simulink model "Inverter_pq_comp_sim"  (R2023b)
settings: Solver=FixedStepDiscrete  StartTime=0.0  StopTime=2  RelTol=1e-3  EnableMultiTasking=on
InitFcn:
  | %% Definition of the parameters
  | 
  | Parameter_Definition
  | 
  | %% Damping
  | 
  | Rd = 3.9;
  | 
  | %% PRes Gains Calculation
  | 
  | % Definicao das grandezas
  | w_cl = 1j*2*pi*1200;  % Phase Crossing Frequency
  | no   = 1;           % Integral Resonant Constant
  | A    = 1;             % Carrier Amplitude
  | 
  | % Kp calculation
  | a0 = 1;
  | a1 = Rd*Cf;
  | b0 = 0;
  | b1 = Lf+Lg;
  | b2 = Rd*Lf*Cf+Rd*Lg*Cf;
  | b3 = Lf*Lg*Cf;
  | 
  | G_lcl = (a1*w_cl+a0)/(b3*w_cl^3+b2*w_cl^2+b1*w_cl+b0);
  | % G_lcl = 1/((Lf+Lg)*w_cl+Rf);
  | 
  | G_PWM = (1/A)*(1-w_cl*Ts/4)/(1+w_cl*Ts/4);
  | 
  | G_wc  = (Vdc/2)*(1/I_base)*G_lcl*G_PWM;
  | 
  | G_wc_abs = abs(G_wc);
  | 
  | Kp = 0.8/G_wc_abs;
  | 
  | % Discretized Controller Gains
  | ressonance_list = [1,5,7];
  | 
  | n_res = length(ressonance_list);
  | a = zeros(2,n_res);
  | b = zeros(2,n_res);
  | Ki_res = zeros(1,n_res);
  | 
  | % for i = 1:n_res
  | %   k = ressonance_list(i);
  | %   Ki_res(i) = (2.2*Kp)/(no*T_gr);
  | %   a(i) = (2*Ki_res(i)*Ts)/(4+((k*w_gr)^2)*Ts^2);
  | %   b(i) = (-8+2*((k*w_gr)^2)*Ts^2)/(4+((k*w_gr)^2)*Ts^2);
  | % end
  | 
  | % wc is the cutoff frequency/damping factor in rad/s
  | wc = 5;
  | 
  | for i = 1:n_res
  |   k = ressonance_list(i);
  |   wk = k * w_gr; % Resonant frequency for this harmonic
  | 
  |   Ki_res(i) = (2.2*Kp)/(0.8*no*T_gr);
  | 
  |   % 1. Calculate the common denominator
  |   den = 4 + 4*wc*Ts + (wk^2)*(Ts^2);
  | ... (+14 lines)
values from neighbouring files (symbols this model uses):
  a1_sogi = single(2*(w0_sogi^2-c_sogi^2)/den0_sogi)    [Parameter_Definition.m]
  a2_sogi = single((c_sogi^2                 - k_sogi*w0_sogi*c_sogi                 + w0_sogi^2)/den0_sogi)    [Parameter_Definition.m]
  bD_sogi = single(k_sogi*w0_sogi*c_sogi/den0_sogi)    [Parameter_Definition.m]
  bQ_sogi = single(k_sogi*w0_sogi^2/den0_sogi)    [Parameter_Definition.m]
  Cdc = 1.5e-3    (= 0.0015)    [Parameter_Definition.m]
  Cf = 5e-6    (= 5e-06)    [Parameter_Definition.m]
  f_gr = 60    [Parameter_Definition.m]
  I_base = S_base/(sqrt(3)*V_gr)    [Parameter_Definition.m]
  Lf = 1e-3    (= 0.001)    [Parameter_Definition.m]
  Lg = 0.5e-3    (= 0.0005)    [Parameter_Definition.m]
  Rdc = 0.1/(2*pi*60*Cdc)    (= 0.176838825658)    [Parameter_Definition.m]
  Rf = 0.1*Xf    (= 0.0376991118431)    [Parameter_Definition.m]
  Rg = 0.1*Xg    (= 0.0188495559215)    [Parameter_Definition.m]
  S_base = S_rated    (= 1000)    [Parameter_Definition.m]
  Ts = 2*(4167)/100e6    (= 8.334e-05)    [Parameter_Definition.m]
  Tstep = Ts/1000    (= 8.334e-08)    [Parameter_Definition.m]
  V_base = sqrt(3)*V_gr    [Parameter_Definition.m]
  V_gr = 127    [Parameter_Definition.m]
  Vdc = 800    [Parameter_Definition.m]
  Vdc_base = Vdc    (= 800)    [Parameter_Definition.m]
  w_gr = 2*pi*f_gr    (= 376.991118431)    [Parameter_Definition.m]
libraries: spsSeriesRLCBranchLib x14, spsIGBTDiodeLib x12, spsCurrentMeasurementLib x6, spsVoltageMeasurementLib x5, c2837xDlib x4, spsACVoltageSourceLib x3, spsGroundLib x3, spsDCVoltageSourceLib x2, spsTriangleGeneratorLib x1, simulink x1, spsThreePhaseBreakerLib x1, sps_lib x1
(part 2 of 2)

== matlab function Inverter_pq_comp_sim/Current Controller/PRes ==
  data: Kp input; a input; b input; errora input; ma output; errorb input; mb output; enable input
function [ma, mb] = PResCurrent(Kp, a, b, errora, errorb, enable)

%Controller modeled in abc frame, considering p.u. values

%%% Variables Definition
%%%%#########################################################
%%%%######################################################### 

nRes = length(a);

max_pu = single(1.0);

%Proportional part variable
%Phase a
persistent pia
    if isempty(pia)
        pia = single(0.0);
    end
%Phase b    
persistent pib
    if isempty(pib)
        pib = single(0.0);
    end 
    
%Resonant parts variables
%Phase a
persistent presa
    if isempty(presa)
        presa = zeros(1,nRes);
    end
persistent presa_1d %1 sample delay
    if isempty(presa_1d)
        presa_1d = zeros(1,nRes);
    end    
persistent presa_2d %2 samples delay
    if isempty(presa_2d)
        presa_2d = zeros(1,nRes);
    end
persistent presOUT_ia
    if isempty(presOUT_ia)
        presOUT_ia = single(0.0);
    end
    
%Phase b
persistent presb
    if isempty(presb)
        presb = zeros(1,nRes);
    end
persistent presb_1d %1 sample delay
    if isempty(presb_1d)
        presb_1d = zeros(1,nRes);
    end    
persistent presb_2d %2 samples delay
    if isempty(presb_2d)
        presb_2d = zeros(1,nRes);
    end
persistent presOUT_ib
    if isempty(presOUT_ib)
        presOUT_ib = single(0.0);
    end

%Error variables
%Phase a
% persistent errora %Actual error
%     if isempty(errora)
%         errora = 0.0;
%     end
persistent errora_0d %Actual error to delay
    if isempty(errora_0d)
        errora_0d = single(0.0);
    end
persistent errora_1d %1 sample delay
    if isempty(errora_1d)
        errora_1d = single(0.0);
    end    
persistent errora_2d %2 sample delay
    if isempty(errora_2d)
        errora_2d = single(0.0);
    end   
%Phase b
% persistent errorb %Actual error
%     if isempty(errorb)
%         errorb = 0.0;
%     end
persistent errorb_0d %Actual error to delay
    if isempty(errorb_0d)
        errorb_0d = single(0.0);
    end
persistent errorb_1d %1 sample delay
    if isempty(errorb_1d)
        errorb_1d = single(0.0);
    end    
persistent errorb_2d %2 sample delay
    if isempty(errorb_2d)
        errorb_2d = single(0.0);
    end

%%% Enable logic
%%%%#########################################################
%%%%#########################################################

if ~enable 
    % Define safe outputs
    ma = single(0.0);
    mb = single(0.0);
    mc = single(0.0);
    
    % Reset history registers for bumpless transfer
    pia = single(0.0); pib = single(0.0);
    
    presa       = zeros(1,nRes);
    presa_1d    = zeros(1,nRes);
    presa_2d    = zeros(1,nRes);
    presOUT_ia  = single(0.0);
    
    presb       = zeros(1,nRes);
    presb_1d    = zeros(1,nRes);
    presb_2d    = zeros(1,nRes);
    presOUT_ib  = single(0.0);
    
    errora_0d = single(0.0); errora_1d = single(0.0); errora_2d = single(0.0);
    errorb_0d = single(0.0); errorb_1d = single(0.0); errorb_2d = single(0.0);
    
    % Exit the function completely
    return; 
end

%%% PRes Current Controllers
%%%%#########################################################
%%%%#########################################################

%Proportional part
pia = errora*Kp;
pib = errorb*Kp;
    
    %Saturation - a
    if pia > max_pu 
        pia = max_pu;
    end
    if pia < -1*max_pu
        pia = -1*max_pu;
    end
    %Saturation - b
    if pib > max_pu
        pib = max_pu;
    end
    if pib < -1*max_pu
        pib = -1*max_pu;
    end   
    
    % %Anti-windup - a
    % if pia > 0.0
    %     limit_ia = max_pu - pia;
    % else
    %     limit_ia = 1 + pia;
    % end
    %  %Anti-windup - b
    % if pib > 0.0
    %     limit_ib = max_pu - pib;
    % else
    %     limit_ib = 1 + pib;
    % end
%     %Anti-windup - c
%     if pic > 0.0
%         limit_ic = max_pu - pic;
%     else
%         limit_ic = 1 + pic;
%     end    
    
    
%Resonant part
errora_2d = errora_1d;
errora_1d = errora_0d;
errora_0d = errora;

errorb_2d = errorb_1d;
errorb_1d = errorb_0d;
errorb_0d = errorb;
        
for i=1:nRes

    %leg a
    presa_2d(i) = presa_1d(i);
	presa_1d(i) = presa(i);
	presa(i) = a(1,i)*errora + a(2,i)*errora_2d - b(1,i)*presa_1d(i) - b(2,i)*presa_2d(i);    
    % if presa(i) > limit_ia
    %     presa(i) = limit_ia;
    % end
    % if presa(i) < -1*limit_ia
    %     presa(i) = -1*limit_ia;
    % end
 
    %leg b
    presb_2d(i) = presb_1d(i);
	presb_1d(i) = presb(i);
	presb(i) = a(1,i)*errorb + a(2,i)*errorb_2d - b(1,i)*presb_1d(i) - b(2,i)*presb_2d(i);    
    % if presb(i) > limit_ib
    %     presb(i) = limit_ib;
    % end
    % if presb(i) < -1*limit_ib
    %     presb(i) = -1*limit_ib;
    % end  
    
end

presOUT_ia = pia;
presOUT_ib = pib;

for i=1:nRes
    presOUT_ia = presOUT_ia + presa(i);
    presOUT_ib = presOUT_ib + presb(i);  
end

%Output for PWM
ma = presOUT_ia;
        %Saturation - ta
        if ma > max_pu 
            ma = max_pu;
        end
        if ma < -1*max_pu
            ma = -1*max_pu;
        end

mb = presOUT_ib;
        %Saturation - tb
        if mb > max_pu 
            mb = max_pu;
        end
        if mb < -1*max_pu
            mb = -1*max_pu;
        end
        
end

== matlab function Inverter_pq_comp_sim/Current Controller/MATLAB Function2 ==
  data: alpha input; a output; beta input; b output; c output; aux output
function [a, b, c, aux] = abc(alpha, beta)

a = sqrt(2/3)*alpha;
b = sqrt(2/3)*(-1*alpha/2 + sqrt(3)*beta/2);
c = sqrt(2/3)*(-1*alpha/2 - sqrt(3)*beta/2);

max_mod = max(abs([a, b, c]));

if max_mod > 1
    scale = 1/max_mod;

    a = a*scale;
    b = b*scale;
    c = c*scale;

    aux = single(1.0);
else
    aux = single(1.0);
end

== matlab function Inverter_pq_comp_sim/MATLAB Function3 ==
  data: a input; alpha output; b input; c input; beta output
function [alpha, beta] = alpha_beta(a, b, c)

alpha = sqrt(2/3)*(a - b/2 - c/2);
beta  = sqrt(2/3)*(sqrt(3)*b/2 - sqrt(3)*c/2);

== matlab function Inverter_pq_comp_sim/pq Current/MATLAB Function ==
  data: p input; i_alpha output; q input; i_beta output; V_alpha input; V_beta input
function [i_alpha, i_beta] = pq_to_i(p, q, V_alpha, V_beta)

i_alpha = (1/(V_alpha^2+V_beta^2))*(V_alpha*p + V_beta*q);
i_beta  = (1/(V_alpha^2+V_beta^2))*(V_beta*p - V_alpha*q);

== matlab function Inverter_pq_comp_sim/Compensation Reference/MATLAB Function ==
  data: i_alpha input; THDi output; i_beta input; v_alpha input; v_beta input; p_EV input; p_avg input; q_avg input
function THDi = THD_calc( ...
    i_alpha, i_beta, ...
    v_alpha, v_beta, ...
    p_EV, p_avg, q_avg)
%#codegen

    window = 200;
    epsilon = 1e-9;

    persistent buffer_I_total;
    persistent buffer_V;
    persistent sum_I_total;
    persistent sum_V;
    persistent idx;
    persistent count;

    if isempty(idx)
        buffer_I_total = zeros(window,1);
        buffer_V = zeros(window,1);

        sum_I_total = single(0.0);
        sum_V = single(0.0);

        idx = 1;
        count = 0;
    end

    % Load-current magnitude squared
    I_total_inst_sq = i_alpha^2 + i_beta^2;

    % Fundamental PCC-voltage magnitude squared
    V_inst_sq = v_alpha^2 + v_beta^2;

    % Remove oldest samples
    old_I = buffer_I_total(idx);
    old_V = buffer_V(idx);

    % Insert newest samples
    buffer_I_total(idx) = I_total_inst_sq;
    buffer_V(idx) = V_inst_sq;

    % Update moving sums
    sum_I_total = ...
        sum_I_total + I_total_inst_sq - old_I;

    sum_V = ...
        sum_V + V_inst_sq - old_V;

    idx = idx + 1;

    if idx > window
        idx = 1;
    end

    if count < window
        count = count + 1;
    end

    % Do not calculate THD before one complete cycle
    if count < window
        THDi = single(0.0);
        return;
    end

    % Squared total load-current magnitude
    IL_total_sq = max(sum_I_total/window,0);

    % Squared fundamental voltage magnitude
    V1_sq = max(sum_V/window,epsilon);

    % Fundamental LOAD current
    IL_fund_sq = ...
        (p_avg^2 + q_avg^2)/V1_sq;

    % Harmonic LOAD current
    IH_load_sq = max( ...
        IL_total_sq - IL_fund_sq, ...
        0);

    % Fundamental grid current including EV charging
    %
    % Current convention:
    % p_EV is negative during charging.
    p_total_fund = p_avg - p_EV;

    IT_fund_sq = ...
        (p_total_fund^2 + q_avg^2)/V1_sq;

    % Equivalent pre-compensation grid THD
    if IT_fund_sq <= epsilon
        THDi = single(0.0);
    else
        THDi = sqrt(IH_load_sq/IT_fund_sq);
    end
end

== matlab function Inverter_pq_comp_sim/MATLAB Function1 ==
  data: a input; alpha output; b input; c input; beta output
function [alpha, beta] = alpha_beta(a, b, c)

alpha = sqrt(2/3)*(a - b/2 - c/2);
beta  = sqrt(2/3)*(sqrt(3)*b/2 - sqrt(3)*c/2);

== matlab function Inverter_pq_comp_sim/MATLAB Function ==
  data: v_unf input; v_f output; bD input; bQ input; a1 input; a2 input; enable input
function v_f  = SOGI(v_unf, bD, bQ, a1, a2, enable)

persistent u1 u2
persistent vf1 vf2
persistent vq1 vq2

if isempty(u1)
    u1  = single(0);
    u2  = single(0);

    vf1 = single(0);
    vf2 = single(0);

    vq1 = single(0);
    vq2 = single(0);
end

if enable == 0
    u1  = single(0);
    u2  = single(0);

    vf1 = single(0);
    vf2 = single(0);

    vq1 = single(0);
    vq2 = single(0);

    v_f = single(0);
    v_q = single(0);
    return;
end

u   = single(v_unf);
bd  = single(bD);
bq  = single(bQ);
aa1 = single(a1);
aa2 = single(a2);

% In-phase band-pass output
v_f = bd*(u - u2) ...
    - aa1*vf1 ...
    - aa2*vf2;

% Quadrature output
v_q = bq*(u + single(2)*u1 + u2) ...
    - aa1*vq1 ...
    - aa2*vq2;

% Update histories AFTER calculating both outputs
u2 = u1;
u1 = u;

vf2 = vf1;
vf1 = v_f;

vq2 = vq1;
vq1 = v_q;

end

== matlab function Inverter_pq_comp_sim/MATLAB Function4 ==
  data: v_unf input; v_f output; bD input; bQ input; a1 input; a2 input; enable input
function v_f  = SOGI(v_unf, bD, bQ, a1, a2, enable)

persistent u1 u2
persistent vf1 vf2
persistent vq1 vq2

if isempty(u1)
    u1  = single(0);
    u2  = single(0);

    vf1 = single(0);
    vf2 = single(0);

    vq1 = single(0);
    vq2 = single(0);
end

if enable == 0
    u1  = single(0);
    u2  = single(0);

    vf1 = single(0);
    vf2 = single(0);

    vq1 = single(0);
    vq2 = single(0);

    v_f = single(0);
    v_q = single(0);
    return;
end

u   = single(v_unf);
bd  = single(bD);
bq  = single(bQ);
aa1 = single(a1);
aa2 = single(a2);

% In-phase band-pass output
v_f = bd*(u - u2) ...
    - aa1*vf1 ...
    - aa2*vf2;

% Quadrature output
v_q = bq*(u + single(2)*u1 + u2) ...
    - aa1*vq1 ...
    - aa2*vq2;

% Update histories AFTER calculating both outputs
u2 = u1;
u1 = u;

vf2 = vf1;
vf1 = v_f;

vq2 = vq1;
vq1 = v_q;

end

== matlab function Inverter_pq_comp_sim/MATLAB Function2 ==
  data: a input; alpha output; b input; c input; beta output
function [alpha, beta] = alpha_beta(a, b, c)

alpha = sqrt(2/3)*(a - b/2 - c/2);
beta  = sqrt(2/3)*(sqrt(3)*b/2 - sqrt(3)*c/2);

== matlab function Inverter_pq_comp_sim/RMS_fcn ==
  data: RMSin input; yout output
function yout = fcn(RMSin)

win = 200;

persistent sampleRMS
    if isempty(sampleRMS)
        sampleRMS = single(0.0);
    end
    if sampleRMS>=win
        sampleRMS = single(0.0);
    end

persistent RMSout
if isempty(RMSout)
    RMSout = single(0.0);
end    
persistent sumRMS
if isempty(sumRMS)
    sumRMS = single(0.0);
end
persistent RMSinArray
     if isempty(RMSinArray)
         RMSinArray = zeros(1,win);
     end

sampleRMS = sampleRMS + 1;      

%RMS of Input Signal
sumRMS = sumRMS + RMSin*RMSin - RMSinArray(1,sampleRMS);
RMSinArray(1,sampleRMS) = RMSin*RMSin;
if sumRMS>=0.0
    RMSout = sqrt(sumRMS/win);
end

%RMSout = RMSout_temp;

yout = RMSout;

== matlab function Inverter_pq_comp_sim/RMS_fcn1 ==
  data: RMSin input; yout output
function yout = fcn(RMSin)

win = 200;

persistent sampleRMS
    if isempty(sampleRMS)
        sampleRMS = single(0.0);
    end
    if sampleRMS>=win
        sampleRMS = single(0.0);
    end

persistent RMSout
if isempty(RMSout)
    RMSout = single(0.0);
end    
persistent sumRMS
if isempty(sumRMS)
    sumRMS = single(0.0);
end
persistent RMSinArray
     if isempty(RMSinArray)
         RMSinArray = zeros(1,win);
     end

sampleRMS = sampleRMS + 1;      

%RMS of Input Signal
sumRMS = sumRMS + RMSin*RMSin - RMSinArray(1,sampleRMS);
RMSinArray(1,sampleRMS) = RMSin*RMSin;
if sumRMS>=0.0
    RMSout = sqrt(sumRMS/win);
end

%RMSout = RMSout_temp;

yout = RMSout;

== matlab function Inverter_pq_comp_sim/RMS_fcn2 ==
  data: RMSin input; yout output
function yout = fcn(RMSin)

win = 200;

persistent sampleRMS
    if isempty(sampleRMS)
        sampleRMS = single(0.0);
    end
    if sampleRMS>=win
        sampleRMS = single(0.0);
    end

persistent RMSout
if isempty(RMSout)
    RMSout = single(0.0);
end    
persistent sumRMS
if isempty(sumRMS)
    sumRMS = single(0.0);
end
persistent RMSinArray
     if isempty(RMSinArray)
         RMSinArray = zeros(1,win);
     end

sampleRMS = sampleRMS + 1;      

%RMS of Input Signal
sumRMS = sumRMS + RMSin*RMSin - RMSinArray(1,sampleRMS);
RMSinArray(1,sampleRMS) = RMSin*RMSin;
if sumRMS>=0.0
    RMSout = sqrt(sumRMS/win);
end

%RMSout = RMSout_temp;

yout = RMSout;

== matlab function Inverter_pq_comp_sim/RMS_fcn3 ==
  data: RMSin input; yout output
function yout = fcn(RMSin)

win = 200;

persistent sampleRMS
    if isempty(sampleRMS)
        sampleRMS = single(0.0);
    end
    if sampleRMS>=win
        sampleRMS = single(0.0);
    end

persistent RMSout
if isempty(RMSout)
    RMSout = single(0.0);
end    
persistent sumRMS
if isempty(sumRMS)
    sumRMS = single(0.0);
end
persistent RMSinArray
     if isempty(RMSinArray)
         RMSinArray = zeros(1,win);
     end

sampleRMS = sampleRMS + 1;      

%RMS of Input Signal
sumRMS = sumRMS + RMSin*RMSin - RMSinArray(1,sampleRMS);
RMSinArray(1,sampleRMS) = RMSin*RMSin;
if sumRMS>=0.0
    RMSout = sqrt(sumRMS/win);
end

%RMSout = RMSout_temp;

yout = RMSout;
